simulink model "untitled1"  (R2024b)
settings: Solver=FixedStepAuto  StartTime=0.0  StopTime=15.0  FixedStep=0.01  RelTol=1e-3
settings Model: Creator=andrey  LastModifiedBy=andrey

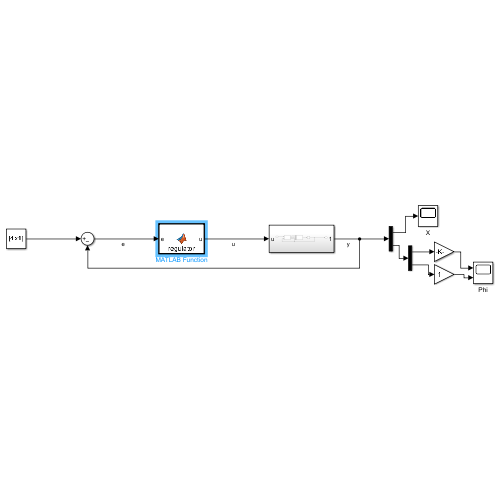
[thumbnail: Simulink's stored preview of the top-level diagram]
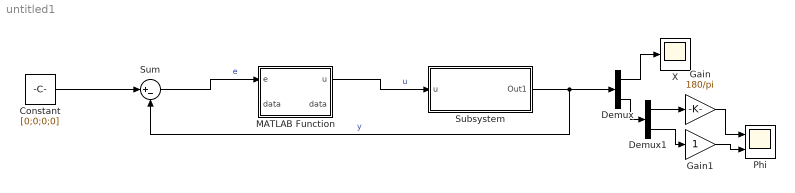
== system untitled1 ==
  Constant : Constant  Value=[0;0;0;0]
  Demux : Demux  Outputs=2
  Demux1 : Demux  Outputs=2
  Gain : Gain  Gain=180/pi
  Gain1 : Gain
  MATLAB Function : MATLAB Function  TreatAsAtomicUnit=on
  Phi : Scope  NumInputPorts=2
  Subsystem : Subsystem
  Sum : Sum  Inputs=|+-
  X : Scope
  wires:
  MATLAB Function/1(u) -> Subsystem/1(u)  "u"
  Subsystem/1(Out1) -> Demux/1, Sum/2  "y"
  Constant/1 -> Sum/1
  Sum/1 -> MATLAB Function/1(e)  "e"
  Demux/1 -> X/1
  Demux1/1 -> Gain/1
  Demux1/2 -> Gain1/1
  Demux/2 -> Demux1/1
  Gain/1 -> Phi/1
  Gain1/1 -> Phi/2

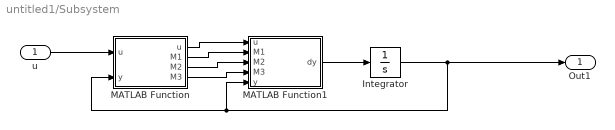
== system untitled1/Subsystem ==
  u : Inport
  Integrator : Integrator  InitialCondition=[0;0;2*pi/180;0]
  MATLAB Function : MATLAB Function  TreatAsAtomicUnit=on
  MATLAB Function1 : MATLAB Function  TreatAsAtomicUnit=on
  Out1 : Outport
  wires:
  u/1 -> MATLAB Function/1("u ")
  MATLAB Function/1(u) -> MATLAB Function1/1(u)
  MATLAB Function/2(M1) -> MATLAB Function1/2(M1)
  MATLAB Function/3(M2) -> MATLAB Function1/3(M2)
  MATLAB Function/4(M3) -> MATLAB Function1/4(M3)
  MATLAB Function1/1(dy) -> Integrator/1
  Integrator/1 -> MATLAB Function/2(y), MATLAB Function1/5(y), Out1/1

== matlab function untitled1/Subsystem/MATLAB Function1 ==
  data: u input; M1 input; M2 input; M3 input; dy output; y input
function dy = rightParts(u, M1, M2, M3, y)
    Fsopr = 0;
    Fpr = 0;
    Fupr = u;
    l = 0.15;
    b2 = 0.01;
    k2 = 0;
    g = 9.8;

    M = [1 0 0 0;
        0 1 0 -(M2*l*cos(y(3)))/M1;
        0 0 1 0;
        0 -(M2 * l *cos(y(3)))/(M3* l^2) 0 1
        ];
    A = [y(2); (Fupr - Fsopr - Fpr - M2*l*(y(4) ^ 2)* sin(y(3)))/M1; y(4); (M2*g*l*sin(y(3)) - b2*y(4) - k2*y(3))/(M3* l^2)];

    dy = M \ A;

== matlab function untitled1/Subsystem/MATLAB Function ==
  data: u input; u output; y input; M1 output; M2 output; M3 output
function [u, M1, M2, M3] = updatedVariabels(u, y)
    m1 = 0.5;
    m2 = 0.15; 
    m3 = 0.05;
    
    M1 = m1 + m2 + m3;
    M2 = m2 + 0.5 * m3;
    M3 = m2 + m3 / 3;

== matlab function untitled1/MATLAB Function ==
  settings: updateMethod=DISCRETE
  data: u output; e input; data input; data output
function [u, data] = regulator(e, data)
    Kp = [0; 0; 0];
    Ki = 0;
    dt = 0.01;
    ei = ei + e(3) * dt;
    data = e(1);
    u = Kp(1) * e(1) + Kp(2) * e(2) + Kp(3) * e(3) ;
